simulink model "Powertrain_Comparison"  (R2024b)
settings: Solver=FixedStepDiscrete  StartTime=0.0  StopTime=3600  FixedStep=1  RelTol=1e-3
InitFcn:
  | try; sc=find_system(bdroot,'LookUnderMasks','all','FollowLinks','on','BlockType','Scope'); for k=1:numel(sc); c=get_param(sc{k},'ScopeConfiguration'); try; c.AxesScaling='Auto'; catch; end; try; nd=prod(c.LayoutDimensions); catch; nd=1; end; for d=1:nd; try; c.ActiveDisplay=d; catch; end; try; c.ShowLegend=true; catch; end; end; end; catch; end
(part 1 of 4)
Description:
  | Standalone requested-speed fuel-cell/battery and diesel energy comparison. Repaired with native MATLAB R2024b block ports and connections. Component data remain study assumptions.
settings Model: Creator=Bless Kofi Atisu  LastModifiedBy=Kuami-Neymar
settings ConfigSet: Description=Self-contained HiAce comparison; discrete one-second simulation
settings SolverCC: AlgebraicLoopSolver=TrustRegion
settings DataIOCC: ExternalInput=[]  InitialState=[]  VisualizeSimOutput=off
settings DebuggingCC: SignalInfNanChecking=error  UnconnectedInputMsg=error  UnconnectedOutputMsg=error  UnconnectedLineMsg=error
settings ModelReferenceCC: EnableRefExpFcnMdlSchedulingChecks=on
settings RTWCC: GPUComputeCapability=3.5  DLArmComputeVersion=19.05

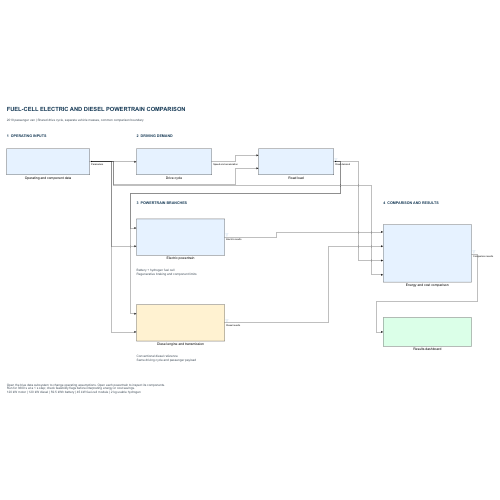
[thumbnail: Simulink's stored preview of the top-level diagram]
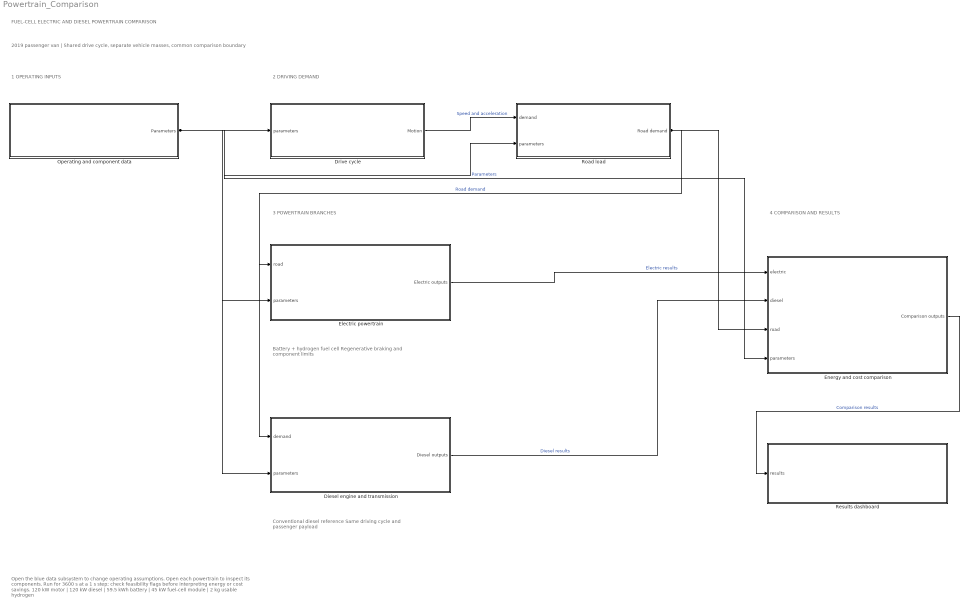
== system Powertrain_Comparison ==
  note: FUEL-CELL ELECTRIC AND DIESEL POWERTRAIN COMPARISON
  note: 2019 passenger van | Shared drive cycle, separate vehicle masses, common comparison boundary
  note: 1 OPERATING INPUTS
  note: 2 DRIVING DEMAND
  note: 3 POWERTRAIN BRANCHES
  note: 4 COMPARISON AND RESULTS
  note: Battery + hydrogen fuel cell
      | Regenerative braking and component limits
  note: Conventional diesel reference
      | Same driving cycle and passenger payload
  note: Open the blue data subsystem to change operating assumptions. Open each powertrain to inspect its components.
      | Run for 3600 s at a 1 s step; check feasibility flags before interpreting energy or cost savings.
      | 120 kW motor | 120 kW diesel | 59.5 kWh battery | 45 kW fuel-cell module | 2 kg usable hydrogen
  Diesel engine and transmission : Subsystem
  Drive cycle : Subsystem
  Electric powertrain : Subsystem
  Energy and cost comparison : Subsystem
  Operating and component data : Subsystem
  Results dashboard : Subsystem
  Road load : Subsystem
  wires:
  Diesel engine and transmission/1(Diesel outputs) -> Energy and cost comparison/2(diesel)  "Diesel results"
  Operating and component data/1(Parameters) -> Road load/2(parameters), Energy and cost comparison/4(parameters), Electric powertrain/2(parameters), Diesel engine and transmission/2(parameters), Drive cycle/1(parameters)  "Parameters"
  Drive cycle/1(Motion) -> Road load/1(demand)  "Speed and acceleration"
  Road load/1(Road demand) -> Energy and cost comparison/3(road), Electric powertrain/1(road), Diesel engine and transmission/1(demand)  "Road demand"
  Energy and cost comparison/1(Comparison outputs) -> Results dashboard/1(results)  "Comparison results"
  Electric powertrain/1(Electric outputs) -> Energy and cost comparison/1(electric)  "Electric results"

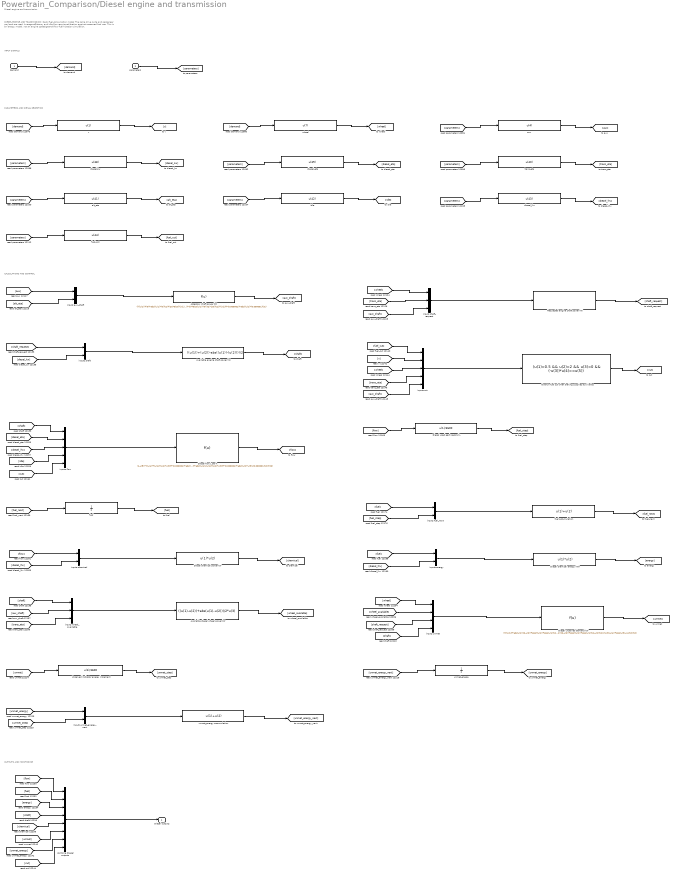
== system Powertrain_Comparison/Diesel engine and transmission ==
  note: Diesel engine and transmission
  note: DIESEL ENGINE AND TRANSMISSION | basic fuel-consumption model
      | The same drive cycle and passenger payload are used. Average efficiency and idle flow require calibration against measured
      | fuel use.
      | This is an energy model, not an engine speed/gear-shift or fuel-injection simulation.
  note: INPUT SIGNALS
  note: PARAMETERS AND SIGNAL SELECTION
  note: CALCULATIONS AND CONTROL
  note: OUTPUTS AND MONITORING
  demand : Inport  PortDimensions=9
  parameters : Inport  Port=2  PortDimensions=52
  Accessory shaft power kW : Fcn  Expr=(((((u(1))+(0)+abs((u(1))-(0)))/2)+(20)-abs((((u(1))+(0)+abs((u(1))-(0)))/2)-(20)))/2)/(((u(2))+(0.000001)+abs((u(2))-(0.000001)))/2)
  Available diesel wheel power kW : Fcn  Expr=((u(1)-u(2))+abs(u(1)-u(2)))/2*u(3)
  Available engine shaft power kW : Fcn  Expr=((u(1))+(u(2))-abs((u(1))-(u(2))))/2
  Diesel chemical energy kWh : Fcn  Expr=u(1)*u(2)
  Diesel chemical power kW : Fcn  Expr=u(1)*u(2)
  Diesel flow L per h : Fcn  Expr=(1-u(5))*(((u(4))+(u(1)/(((u(2)*u(3))+(0.000001)+abs((u(2)*u(3))-(0.000001)))/2))+abs((u(4))-(u(1)/(((u(2)*u(3))+(0.000001)+abs((u(2)*u(3))-(0.000001)))/2))))/2)
  Diesel unserved demand kW : Fcn  Expr=((((((u(1))+abs(u(1)))/2-u(2))+abs(((u(1))+abs(u(1)))/2-u(2)))/2)+(((u(3)-u(4))+abs(u(3)-u(4)))/2)+abs((((((u(1))+abs(u(1)))/2-u(2))+abs(((u(1))+abs(u(1)))/2-u(2)))/2)-(((u(3)-u(4))+abs(u(3)-u(4)))/2)))/2
  Diesel used each second L : Fcn  Expr=u(1)/3600
  Overrun fuel cut when braking supplies auxiliaries : Fcn  Expr=(u(1)>0.5 && u(2)>2 && u(3)<0 && (-u(3))*u(4)>=u(5))
  Requested engine shaft power kW : Fcn  Expr=(((u(1))+abs(u(1)))/2)/(((u(2))+(0.000001)+abs((u(2))-(0.000001)))/2)+u(3)
  Unserved indicator energy increment : Fcn  Expr=u(1)/3600
  alt_eta : Fcn  Expr=u(41)
  aux : Fcn  Expr=u(4)
  combine Diesel outputs : Mux  Inputs=8
  diesel_eta : Fcn  Expr=u(39)
  diesel_kw : Fcn  Expr=u(38)
  diesel_lhv : Fcn  Expr=u(43)
  fuel : UnitDelay
  fuel accumulation : Fcn  Expr=u(1)+u(2)
  fuel_cut : Fcn  Expr=u(44)
  idle : Fcn  Expr=u(42)
  inputs aux_shaft : Mux  Inputs=2
  inputs chemical : Mux  Inputs=2
  inputs cut : Mux  Inputs=5
  inputs energy : Mux  Inputs=2
  inputs flow : Mux  Inputs=5
  inputs fuel_next : Mux  Inputs=2
  inputs shaft : Mux  Inputs=2
  inputs shaft_request : Mux  Inputs=3
  inputs unmet : Mux
  inputs unmet_energy_next : Mux  Inputs=2
  inputs wheel_available : Mux  Inputs=3
  trans_eta : Fcn  Expr=u(40)
  unmet_energy : UnitDelay
  unmet_energy accumulation : Fcn  Expr=u(1)+u(2)
  v : Fcn  Expr=u(1)
  wheel : Fcn  Expr=u(7)
  Diesel outputs : Outport  PortDimensions=8
  wires:
  [parameters] -> trans_eta/1
  Accessory shaft power kW/1 -> [aux_shaft]
  [parameters] -> idle/1
  [shaft] -> inputs wheel_available/1
  [parameters] -> fuel_cut/1
  [diesel_lhv] -> inputs chemical/2
  [flow] -> inputs chemical/1
  [fuel] -> inputs fuel_next/1
  [energy] -> combine Diesel outputs/3
  [diesel_lhv] -> inputs energy/2
  [flow] -> Diesel used each second L/1
  [diesel_lhv] -> inputs flow/3
  [flow] -> combine Diesel outputs/1
  [parameters] -> diesel_kw/1
  [fuel_next] -> fuel/1
  [idle] -> inputs flow/4
  [fuel] -> combine Diesel outputs/2
  [trans_eta] -> inputs cut/4
  [unmet] -> Unserved indicator energy increment/1
  Overrun fuel cut when braking supplies auxiliaries/1 -> [cut]
  [shaft_request] -> inputs unmet/3
  [shaft] -> combine Diesel outputs/4
  [diesel_kw] -> inputs shaft/2
  [demand] -> wheel/1
  [cut] -> combine Diesel outputs/8
  [chemical] -> combine Diesel outputs/5
  [wheel] -> inputs shaft_request/1
  [unmet_step] -> inputs unmet_energy_next/2
  [unmet] -> combine Diesel outputs/6
  [unmet_energy] -> combine Diesel outputs/7
  parameters/1 -> [parameters]
  [parameters] -> diesel_lhv/1
  [parameters] -> alt_eta/1
  [parameters] -> diesel_eta/1
  [shaft] -> inputs flow/1
  demand/1 -> [demand]
  [demand] -> v/1
  [aux_shaft] -> inputs wheel_available/2
  [cut] -> inputs flow/5
  [diesel_eta] -> inputs flow/2
  [trans_eta] -> inputs shaft_request/2
  [shaft_request] -> inputs shaft/1
  [shaft] -> inputs unmet/4
  [trans_eta] -> inputs wheel_available/3
  Diesel chemical energy kWh/1 -> [energy]
  [fuel] -> inputs energy/1
  [fuel_cut] -> inputs cut/1
  [parameters] -> aux/1
  [fuel_step] -> inputs fuel_next/2
  inputs unmet/1 -> Diesel unserved demand kW/1
  [wheel] -> inputs unmet/1
  inputs fuel_next/1 -> fuel accumulation/1
  inputs shaft_request/1 -> Requested engine shaft power kW/1
  [wheel_available] -> inputs unmet/2
  [wheel] -> inputs cut/3
  [v] -> inputs cut/2
  Diesel unserved demand kW/1 -> [unmet]
  [unmet_energy] -> inputs unmet_energy_next/1
  [unmet_energy_next] -> unmet_energy/1
  [aux_shaft] -> inputs cut/5
  unmet_energy/1 -> [unmet_energy]
  [aux] -> inputs aux_shaft/1
  [aux_shaft] -> inputs shaft_request/3
  [alt_eta] -> inputs aux_shaft/2
  fuel_cut/1 -> [fuel_cut]
  combine Diesel outputs/1 -> Diesel outputs/1
  inputs flow/1 -> Diesel flow L per h/1
  diesel_eta/1 -> [diesel_eta]
  inputs wheel_available/1 -> Available diesel wheel power kW/1
  fuel/1 -> [fuel]
  wheel/1 -> [wheel]
  diesel_kw/1 -> [diesel_kw]
  Unserved indicator energy increment/1 -> [unmet_step]
  inputs unmet_energy_next/1 -> unmet_energy accumulation/1
  aux/1 -> [aux]
  Diesel used each second L/1 -> [fuel_step]
  inputs shaft/1 -> Available engine shaft power kW/1
  v/1 -> [v]
  inputs aux_shaft/1 -> Accessory shaft power kW/1
  idle/1 -> [idle]
  alt_eta/1 -> [alt_eta]
  inputs cut/1 -> Overrun fuel cut when braking supplies auxiliaries/1
  inputs energy/1 -> Diesel chemical energy kWh/1
  inputs chemical/1 -> Diesel chemical power kW/1
  diesel_lhv/1 -> [diesel_lhv]
  trans_eta/1 -> [trans_eta]
  Diesel flow L per h/1 -> [flow]
  Available diesel wheel power kW/1 -> [wheel_available]
  fuel accumulation/1 -> [fuel_next]
  unmet_energy accumulation/1 -> [unmet_energy_next]
  Available engine shaft power kW/1 -> [shaft]
  Diesel chemical power kW/1 -> [chemical]
  Requested engine shaft power kW/1 -> [shaft_request]

== system Powertrain_Comparison/Drive cycle ==
  note: Drive cycle
  note: DRIVE CYCLE | same speed and road inputs for both powertrains
      | Cycle mode: 600 s repeated demonstration, ramp 0-80 s, cruise 80-500 s, brake 500-580 s, stop 580-600 s.
  note: INPUT SIGNALS
  note: PARAMETERS AND SIGNAL SELECTION
  note: CALCULATIONS AND CONTROL
  note: OUTPUTS AND MONITORING
  parameters : Inport  PortDimensions=52
  Acceleration cruise braking stop fraction : Fcn  Expr=(u(1)<80)*u(1)/80+(u(1)>=80 && u(1)<500)+(u(1)>=500 && u(1)<580)*(580-u(1))/80
  Commanded acceleration m per s2 : Fcn  Expr=u(1)-u(2)
  Commanded distance increment km : Fcn  Expr=u(1)/1000
  Cycle time s : Fcn  Expr=rem(u(1),600)
  Interval mean speed m per s : Fcn  Expr=(u(1)+u(2))/2
  Limited commanded speed m per s : Fcn  Expr=u(1)+((((u(2)-u(1))+(-u(4))+abs((u(2)-u(1))-(-u(4))))/2)+(u(3))-abs((((u(2)-u(1))+(-u(4))+abs((u(2)-u(1))-(-u(4))))/2)-(u(3))))/2
  Simulation time : DigitalClock
  Target speed m per s : Fcn  Expr=(((((u(1))+(0)+abs((u(1))-(0)))/2)+(100)-abs((((u(1))+(0)+abs((u(1))-(0)))/2)-(100)))/2)*((u(2)>=0.5)*u(3)+(u(2)<0.5))/3.6
  accel : Fcn  Expr=u(50)
  combine Motion : Mux  Inputs=3
  decel : Fcn  Expr=u(51)
  distance : UnitDelay
  distance accumulation : Fcn  Expr=u(1)+u(2)
  inputs a : Mux  Inputs=2
  inputs distance_next : Mux  Inputs=2
  inputs next_speed : Mux
  inputs target : Mux  Inputs=3
  inputs v : Mux  Inputs=2
  old_speed : UnitDelay
  profile : Fcn  Expr=u(2)
  speed : Fcn  Expr=u(1)
  Motion : Outport  PortDimensions=3
  wires:
  [speed] -> inputs target/1
  [old_speed] -> inputs a/2
  [next_speed] -> inputs v/2
  [parameters] -> decel/1
  [shape] -> inputs target/3
  [parameters] -> accel/1
  [old_speed] -> inputs v/1
  [next_speed] -> old_speed/1
  Simulation time/1 -> [time]
  inputs v/1 -> Interval mean speed m per s/1
  [accel] -> inputs next_speed/3
  [distance_next] -> distance/1
  [v] -> Commanded distance increment km/1
  parameters/1 -> [parameters]
  [distance_step] -> inputs distance_next/2
  [profile] -> inputs target/2
  [old_speed] -> inputs next_speed/1
  [parameters] -> profile/1
  [phase] -> Acceleration cruise braking stop fraction/1
  [target] -> inputs next_speed/2
  [parameters] -> speed/1
  [next_speed] -> inputs a/1
  [decel] -> inputs next_speed/4
  [time] -> Cycle time s/1
  [v] -> combine Motion/1
  [distance] -> combine Motion/3
  [a] -> combine Motion/2
  profile/1 -> [profile]
  [distance] -> inputs distance_next/1
  inputs distance_next/1 -> distance accumulation/1
  decel/1 -> [decel]
  accel/1 -> [accel]
  distance/1 -> [distance]
  old_speed/1 -> [old_speed]
  Commanded distance increment km/1 -> [distance_step]
  inputs a/1 -> Commanded acceleration m per s2/1
  speed/1 -> [speed]
  inputs next_speed/1 -> Limited commanded speed m per s/1
  Cycle time s/1 -> [phase]
  inputs target/1 -> Target speed m per s/1
  distance accumulation/1 -> [distance_next]
  combine Motion/1 -> Motion/1
  Acceleration cruise braking stop fraction/1 -> [shape]
  Interval mean speed m per s/1 -> [v]
  Commanded acceleration m per s2/1 -> [a]
  Limited commanded speed m per s/1 -> [next_speed]
  Target speed m per s/1 -> [target]

== system Powertrain_Comparison/Electric powertrain ==
  note: Electric powertrain
  note: ELECTRIC POWERTRAIN | hydrogen and battery feed the electric motor
      | Battery management is reused from the battery project. Motor and converter equations are adapted from the electric-drive
      | project.
  note: INPUT SIGNALS
  note: CALCULATIONS AND CONTROL
  note: OUTPUTS AND MONITORING
  road : Inport  PortDimensions=9
  parameters : Inport  Port=2  PortDimensions=52
  Ambient temperature : Fcn  Expr=u(5)
  Battery DC converter : Subsystem
  Battery power limits : Subsystem
  Battery storage : Subsystem
  DC boost converter : Subsystem
  DC bus and braking : Subsystem
  Energy management : Subsystem
  Fuel cell module : Subsystem
  Hydrogen storage : Subsystem
  Inverter : Subsystem
  Motor : Subsystem
  combine Electric outputs : Mux  Inputs=9
  Electric outputs : Outport  PortDimensions=51
  wires:
  DC bus and braking/1(Bus signals) -> [balance]
  [motor] -> DC bus and braking/4(motor)
  Motor/1(Motor signals) -> [motor], Inverter/1(demand)
  [inverter] -> DC bus and braking/1(inverter)
  [fc_converter] -> DC bus and braking/2(fc_bus)
  [fuelcell] -> Hydrogen storage/1(demand)
  [battery_actual] -> DC bus and braking/3(battery_actual)
  road/1 -> [road]
  [road] -> DC bus and braking/5(road)
  [parameters] -> DC bus and braking/6(parameters)
  DC boost converter/1(Converter signals) -> [fc_converter]
  [parameters] -> Hydrogen storage/2(parameters)
  Battery DC converter/1(Current command) -> [current]
  [ems] -> Battery DC converter/1(dispatch)
  [fc_converter] -> Battery DC converter/2(fuel_cell_bus)
  [battery_state] -> Battery DC converter/3(battery_state)
  [limits] -> Battery DC converter/4(limits)
  [parameters] -> Battery DC converter/5(parameters)
  [road] -> Motor/1(demand)
  [parameters] -> Motor/2(parameters)
  [inverter] -> Energy management/1(inverter)
  [battery_state] -> Energy management/2(battery)
  [limits] -> Energy management/3(limits)
  [hydrogen] -> Energy management/4(hydrogen)
  [parameters] -> Energy management/5(parameters)
  [hydrogen] -> combine Electric outputs/6
  parameters/1 -> [parameters]
  [battery_state] -> Battery power limits/1(demand)
  [parameters] -> Battery power limits/2(parameters)
  Battery storage/1(Battery state) -> [battery_state]
  [parameters] -> Ambient temperature/1
  [battery_state] -> combine Electric outputs/1
  [battery_actual] -> combine Electric outputs/2
  [motor] -> combine Electric outputs/3
  [inverter] -> combine Electric outputs/4
  [fuelcell] -> combine Electric outputs/5
  [fc_converter] -> combine Electric outputs/7
  [balance] -> combine Electric outputs/8
  [battery_request] -> combine Electric outputs/9
  [current] -> Battery storage/1(current_request)
  Hydrogen storage/1(Inventory) -> [hydrogen]
  Ambient temperature/1 -> Battery storage/2(ambient)
  Battery DC converter/2(Converter request) -> [battery_request]
  Energy management/1(Dispatch) -> [ems], Fuel cell module/1(dispatch)
  [parameters] -> Inverter/2(parameters)
  [hydrogen] -> Fuel cell module/2(hydrogen)
  [parameters] -> Fuel cell module/3(parameters)
  Battery power limits/1(Power limits) -> [limits]
  combine Electric outputs/1 -> Electric outputs/1
  Inverter/1(Inverter signals) -> [inverter]
  Battery storage/2(Battery actual) -> [battery_actual]
  Fuel cell module/1(Fuel cell signals) -> DC boost converter/1(demand), [fuelcell]
  [parameters] -> DC boost converter/2(parameters)

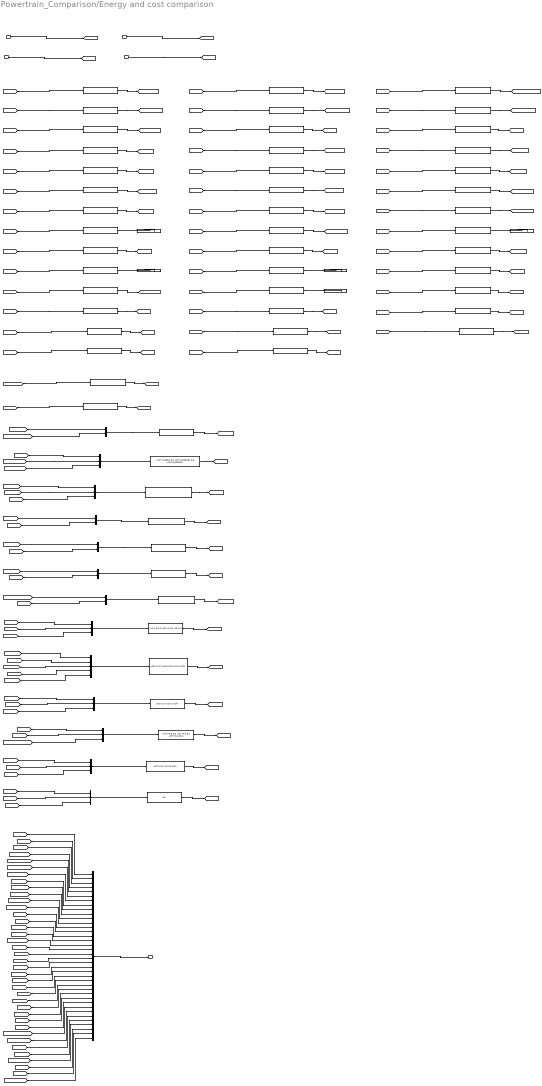
== system Powertrain_Comparison/Energy and cost comparison ==
  note: Energy and cost comparison
  note: ENERGY AND COST COMPARISON | common requested route and payload
      | Net source energy = hydrogen LHV energy + signed battery inventory depletion. Fuel-cell electricity is not counted again.
      | Saving outputs are valid only if both powertrains meet demand. Cost savings also require prices and no battery-energy
      | surplus.
  note: INPUT SIGNALS
  note: PARAMETERS AND SIGNAL SELECTION
  note: CALCULATIONS AND CONTROL
  note: OUTPUTS AND MONITORING
  electric : Inport  PortDimensions=51
  diesel : Inport  Port=2  PortDimensions=8
  road : Inport  Port=3  PortDimensions=9
  parameters : Inport  Port=4  PortDimensions=52
  All energy prices entered 1 yes : Fcn  Expr=(u(1)>0 && u(2)>0 && u(3)>0)
  Battery SOC percent : Fcn  Expr=100*u(1)
  Both powertrains support requested operation 1 yes : Fcn  Expr=(u(1)>0.0001 && u(2)<0.000001 && u(3)<0.000001)
  Calculated diesel litres per 100 km : Fcn  Expr=100*u(1)/(((u(2))+(0.000001)+abs((u(2))-(0.000001)))/2)
  Commanded speed km per h : Fcn  Expr=3.6*u(1)
  Cost saving comparison valid 1 yes : Fcn  Expr=(u(1)>0.5 && u(2)>0.5 && u(3)>=-0.001)
  Diesel refill cost GHS : Fcn  Expr=u(3)*u(1)*u(2)-(1-u(3))
  Energy cost saving GHS -1 unavailable : Fcn  Expr=u(3)*(u(1)-u(2))-(1-u(3))
  Grid recharge energy equivalent kWh : Fcn  Expr=((u(1))+abs(u(1)))/2/(((u(2))+(0.000001)+abs((u(2))-(0.000001)))/2)
  Hydrogen kg per 100 km : Fcn  Expr=100*u(1)/(((u(2))+(0.000001)+abs((u(2))-(0.000001)))/2)
  Hydrogen refill plus recharge cost GHS : Fcn  Expr=u(5)*(u(1)*u(2)+u(3)*u(4))-(1-u(5))
  Mass above study screen kg : Fcn  Expr=((((u(1))+(u(2))+abs((u(1))-(u(2))))/2-u(3))+abs(((u(1))+(u(2))+abs((u(1))-(u(2))))/2-u(3)))/2
  Net onboard source energy kWh : Fcn  Expr=u(1)+u(2)
  Net source energy kWh per 100 km : Fcn  Expr=100*u(1)/(((u(2))+(0.000001)+abs((u(2))-(0.000001)))/2)
  Net source energy saving percent -1 unavailable : Fcn  Expr=u(3)*100*(1-u(1)/(((u(2))+(0.000001)+abs((u(2))-(0.000001)))/2))-(1-u(3))
  Unused diagnostic balance_friction : Terminator
  Unused diagnostic balance_load_energy : Terminator
  Unused diagnostic diesel_chemical : Terminator
  Unused diagnostic diesel_cut : Terminator
  Unused diagnostic diesel_shaft : Terminator
  balance_battery_bus : Fcn  Expr=u(40)
  balance_friction : Fcn  Expr=u(45)
  balance_load_energy : Fcn  Expr=u(47)
  balance_regen_energy : Fcn  Expr=u(48)
  balance_regen_used : Fcn  Expr=u(42)
  balance_unmet : Fcn  Expr=u(41)
  balance_unmet_energy : Fcn  Expr=u(46)
  battery_actual_current : Fcn  Expr=u(14)
  battery_actual_heat : Fcn  Expr=u(18)
  battery_actual_voltage : Fcn  Expr=u(13)
  battery_state_delta_energy : Fcn  Expr=u(10)
  battery_state_nominal : Fcn  Expr=u(8)
  battery_state_soc : Fcn  Expr=u(1)
  battery_state_temp : Fcn  Expr=u(2)
  combine Comparison outputs : Mux  Inputs=38
  diesel_chemical : Fcn  Expr=u(5)
  diesel_cut : Fcn  Expr=u(8)
  diesel_energy : Fcn  Expr=u(3)
  diesel_flow : Fcn  Expr=u(1)
  diesel_fuel : Fcn  Expr=u(2)
  diesel_price : Fcn  Expr=u(47)
  diesel_shaft : Fcn  Expr=u(4)
  diesel_unmet : Fcn  Expr=u(6)
  diesel_unmet_energy : Fcn  Expr=u(7)
  distance : Fcn  Expr=u(3)
  eta_grid : Fcn  Expr=u(48)
  fc_converter_bus : Fcn  Expr=u(37)
  fuelcell_heat : Fcn  Expr=u(33)
  fuelcell_module : Fcn  Expr=u(31)
  grid_price : Fcn  Expr=u(45)
  gross : Fcn  Expr=u(49)
  h2_price : Fcn  Expr=u(46)
  hydrogen_energy : Fcn  Expr=u(36)
  hydrogen_remaining : Fcn  Expr=u(34)
  hydrogen_used : Fcn  Expr=u(35)
  inputs cost_save : Mux  Inputs=3
  inputs cost_valid : Mux  Inputs=3
  inputs diesel_cost : Mux  Inputs=3
  inputs diesel_l100 : Mux  Inputs=2
  inputs energy_save : Mux  Inputs=3
  inputs ev_cost : Mux  Inputs=5
  inputs ev_kwh100 : Mux  Inputs=2
  inputs feasible : Mux  Inputs=3
  inputs grid_recharge : Mux  Inputs=2
  inputs h2_kg100 : Mux  Inputs=2
  inputs mass_excess : Mux  Inputs=3
  inputs net_ev_energy : Mux  Inputs=2
  inputs prices_ready : Mux  Inputs=3
  mass_ev : Fcn  Expr=u(8)
  mass_ice : Fcn  Expr=u(9)
  motor_iq : Fcn  Expr=u(25)
  motor_phase_v : Fcn  Expr=u(26)
  motor_rpm : Fcn  Expr=u(24)
  motor_unmet_motor : Fcn  Expr=u(27)
  v : Fcn  Expr=u(1)
  Comparison outputs : Outport  PortDimensions=38
  wires:
  [ev_cost] -> combine Comparison outputs/27
  [parameters] -> h2_price/1
  motor_rpm/1 -> [motor_rpm]
  [gross] -> inputs mass_excess/3
  [speed_kmh] -> combine Comparison outputs/1
  combine Comparison outputs/1 -> Comparison outputs/1
  balance_battery_bus/1 -> [balance_battery_bus]
  [battery_state_nominal] -> combine Comparison outputs/32
  [balance_regen_energy] -> combine Comparison outputs/38
  Energy cost saving GHS -1 unavailable/1 -> [cost_save]
  battery_state_delta_energy/1 -> [battery_state_delta_energy]
  [diesel_fuel] -> combine Comparison outputs/20
  [fc_converter_bus] -> combine Comparison outputs/10
  [parameters] -> eta_grid/1
  [fuelcell_heat] -> combine Comparison outputs/34
  [h2_kg100] -> combine Comparison outputs/36
  [ev_kwh100] -> combine Comparison outputs/37
  [diesel] -> diesel_fuel/1
  [ev_cost] -> inputs cost_save/2
  [grid_recharge] -> combine Comparison outputs/26
  [soc_percent] -> combine Comparison outputs/3
  inputs ev_cost/1 -> Hydrogen refill plus recharge cost GHS/1
  Hydrogen kg per 100 km/1 -> [h2_kg100]
  [battery_actual_heat] -> combine Comparison outputs/35
  [net_ev_energy] -> combine Comparison outputs/22
  [mass_excess] -> combine Comparison outputs/33
  [hydrogen_remaining] -> combine Comparison outputs/7
  h2_price/1 -> [h2_price]
  [distance] -> combine Comparison outputs/2
  [battery_state_delta_energy] -> combine Comparison outputs/31
  diesel_flow/1 -> [diesel_flow]
  [mass_ev] -> inputs mass_excess/1
  gross/1 -> [gross]
  [cost_valid] -> combine Comparison outputs/30
  [fuelcell_module] -> combine Comparison outputs/9
  [cost_save] -> combine Comparison outputs/29
  balance_unmet_energy/1 -> [balance_unmet_energy]
  [diesel_cost] -> combine Comparison outputs/28
  [diesel_price] -> inputs diesel_cost/2
  [energy_save] -> combine Comparison outputs/24
  [net_ev_energy] -> inputs ev_kwh100/1
  Diesel refill cost GHS/1 -> [diesel_cost]
  mass_ice/1 -> [mass_ice]
  [diesel] -> diesel_cut/1
  [diesel_l100] -> combine Comparison outputs/21
  [balance_regen_used] -> combine Comparison outputs/12
  [electric] -> motor_iq/1
  [battery_actual_voltage] -> combine Comparison outputs/5
  [motor_unmet_motor] -> combine Comparison outputs/17
  [prices_ready] -> inputs diesel_cost/3
  [feasible] -> combine Comparison outputs/25
  balance_load_energy/1 -> Unused diagnostic balance_load_energy/1
  [diesel_unmet] -> combine Comparison outputs/18
  parameters/1 -> [parameters]
  [battery_actual_current] -> combine Comparison outputs/6
  [distance] -> inputs h2_kg100/2
  [battery_state_delta_energy] -> inputs grid_recharge/1
  [diesel_energy] -> combine Comparison outputs/23
  [diesel_flow] -> combine Comparison outputs/19
  diesel/1 -> [diesel]
  [balance_unmet] -> combine Comparison outputs/16
  [motor_phase_v] -> combine Comparison outputs/15
  [motor_iq] -> combine Comparison outputs/14
  balance_regen_used/1 -> [balance_regen_used]
  [battery_state_delta_energy] -> inputs cost_valid/3
  [motor_rpm] -> combine Comparison outputs/13
  [balance_battery_bus] -> combine Comparison outputs/11
  inputs cost_save/1 -> Energy cost saving GHS -1 unavailable/1
  [hydrogen_used] -> combine Comparison outputs/8
  [battery_state_temp] -> combine Comparison outputs/4
  [grid_recharge] -> inputs ev_cost/1
  [diesel] -> diesel_unmet/1
  Mass above study screen kg/1 -> [mass_excess]
  inputs mass_excess/1 -> Mass above study screen kg/1
  [mass_ice] -> inputs mass_excess/2
  [cost_valid] -> inputs cost_save/3
  [diesel_cost] -> inputs cost_save/1
  [battery_state_delta_energy] -> inputs net_ev_energy/2
  Cost saving comparison valid 1 yes/1 -> [cost_valid]
  [diesel_fuel] -> inputs diesel_cost/1
  inputs cost_valid/1 -> Cost saving comparison valid 1 yes/1
  [prices_ready] -> inputs cost_valid/2
  [road] -> mass_ice/1
  [feasible] -> inputs cost_valid/1
  inputs diesel_cost/1 -> Diesel refill cost GHS/1
  [prices_ready] -> inputs ev_cost/5
  Hydrogen refill plus recharge cost GHS/1 -> [ev_cost]
  [h2_price] -> inputs ev_cost/4
  motor_unmet_motor/1 -> [motor_unmet_motor]
  [hydrogen_used] -> inputs ev_cost/3
  [grid_price] -> inputs ev_cost/2
  All energy prices entered 1 yes/1 -> [prices_ready]
  inputs prices_ready/1 -> All energy prices entered 1 yes/1
  [diesel_price] -> inputs prices_ready/3
  [h2_price] -> inputs prices_ready/2
  fuelcell_heat/1 -> [fuelcell_heat]
  [grid_price] -> inputs prices_ready/1
  Grid recharge energy equivalent kWh/1 -> [grid_recharge]
  inputs grid_recharge/1 -> Grid recharge energy equivalent kWh/1
  [eta_grid] -> inputs grid_recharge/2
  [diesel] -> diesel_energy/1
  Net source energy kWh per 100 km/1 -> [ev_kwh100]
  inputs ev_kwh100/1 -> Net source energy kWh per 100 km/1
  [distance] -> inputs ev_kwh100/2
  fc_converter_bus/1 -> [fc_converter_bus]
  inputs h2_kg100/1 -> Hydrogen kg per 100 km/1
  [hydrogen_used] -> inputs h2_kg100/1
  Calculated diesel litres per 100 km/1 -> [diesel_l100]
  inputs diesel_l100/1 -> Calculated diesel litres per 100 km/1
  battery_actual_heat/1 -> [battery_actual_heat]
  [distance] -> inputs diesel_l100/2
  [diesel_fuel] -> inputs diesel_l100/1
  Net source energy saving percent -1 unavailable/1 -> [energy_save]
  inputs energy_save/1 -> Net source energy saving percent -1 unavailable/1
  [feasible] -> inputs energy_save/3
  [diesel_energy] -> inputs energy_save/2
  [net_ev_energy] -> inputs energy_save/1
  Both powertrains support requested operation 1 yes/1 -> [feasible]
  inputs feasible/1 -> Both powertrains support requested operation 1 yes/1
  battery_state_soc/1 -> [battery_state_soc]
  [diesel_unmet_energy] -> inputs feasible/3
  [balance_unmet_energy] -> inputs feasible/2
  [distance] -> inputs feasible/1
  Net onboard source energy kWh/1 -> [net_ev_energy]
  [parameters] -> gross/1
  inputs net_ev_energy/1 -> Net onboard source energy kWh/1
  [hydrogen_energy] -> inputs net_ev_energy/1
  Commanded speed km per h/1 -> [speed_kmh]
  [v] -> Commanded speed km per h/1
  Battery SOC percent/1 -> [soc_percent]
  [battery_state_soc] -> Battery SOC percent/1
  eta_grid/1 -> [eta_grid]
  diesel_price/1 -> [diesel_price]
  [parameters] -> diesel_price/1
  grid_price/1 -> [grid_price]
  [parameters] -> grid_price/1
  mass_ev/1 -> [mass_ev]
  motor_phase_v/1 -> [motor_phase_v]
  [road] -> mass_ev/1
  distance/1 -> [distance]
  [road] -> distance/1
  v/1 -> [v]
  [road] -> v/1
  diesel_cut/1 -> Unused diagnostic diesel_cut/1
  diesel_unmet_energy/1 -> [diesel_unmet_energy]
  [diesel] -> diesel_chemical/1
  [diesel] -> diesel_unmet_energy/1
  diesel_unmet/1 -> [diesel_unmet]
  diesel_chemical/1 -> Unused diagnostic diesel_chemical/1
  electric/1 -> [electric]
  diesel_shaft/1 -> Unused diagnostic diesel_shaft/1
  [diesel] -> diesel_flow/1
  [diesel] -> diesel_shaft/1
  diesel_energy/1 -> [diesel_energy]
  diesel_fuel/1 -> [diesel_fuel]
  balance_friction/1 -> Unused diagnostic balance_friction/1
  [electric] -> balance_friction/1
  balance_regen_energy/1 -> [balance_regen_energy]
  [electric] -> balance_regen_energy/1
  battery_actual_voltage/1 -> [battery_actual_voltage]
  [electric] -> balance_load_energy/1
  motor_iq/1 -> [motor_iq]
  [electric] -> balance_unmet_energy/1
  [electric] -> balance_regen_used/1
  balance_unmet/1 -> [balance_unmet]
  [electric] -> balance_unmet/1
  [electric] -> balance_battery_bus/1
  [electric] -> battery_actual_current/1
  [electric] -> fc_converter_bus/1
  hydrogen_energy/1 -> [hydrogen_energy]
  [electric] -> hydrogen_energy/1
  hydrogen_used/1 -> [hydrogen_used]
  [electric] -> hydrogen_used/1
  hydrogen_remaining/1 -> [hydrogen_remaining]
  [electric] -> hydrogen_remaining/1
  [electric] -> fuelcell_heat/1
  fuelcell_module/1 -> [fuelcell_module]
  [electric] -> fuelcell_module/1
  [electric] -> motor_unmet_motor/1
  [electric] -> motor_phase_v/1
  [electric] -> motor_rpm/1
  [electric] -> battery_actual_heat/1
  battery_actual_current/1 -> [battery_actual_current]
  [electric] -> battery_actual_voltage/1
  battery_state_nominal/1 -> [battery_state_nominal]
  [electric] -> battery_state_nominal/1
  [electric] -> battery_state_delta_energy/1
  battery_state_temp/1 -> [battery_state_temp]
  [electric] -> battery_state_temp/1
  [electric] -> battery_state_soc/1
  road/1 -> [road]

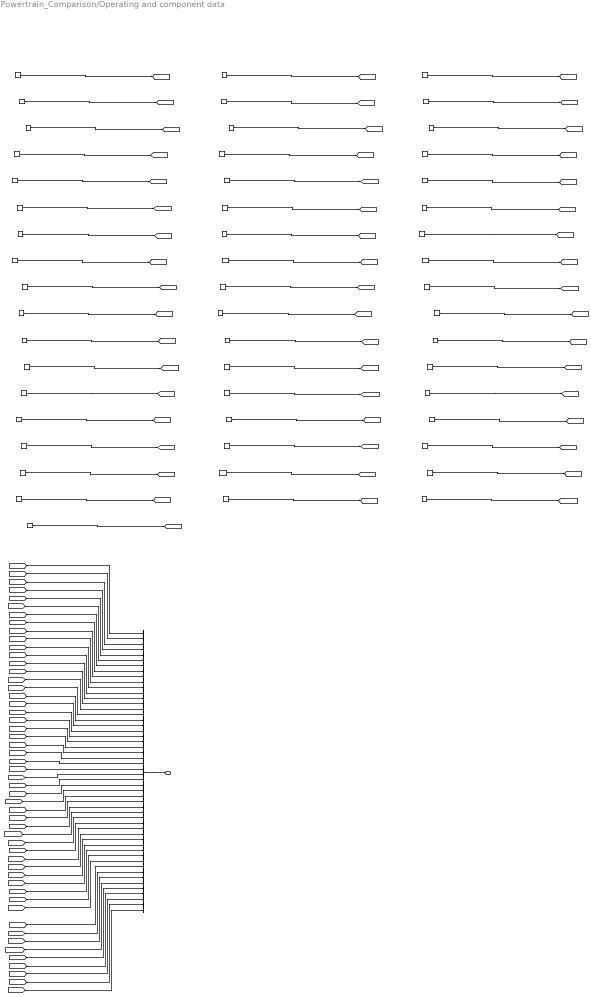
== system Powertrain_Comparison/Operating and component data ==
  note: Operating and component data
  note: ENERGY PRICES
  note: DIESEL ENGINE
  note: FUEL CELL
  note: ELECTRIC DRIVE
  note: VEHICLE DATA
  note: OPERATING CONDITIONS
  note: EDIT PARAMETERS | blue blocks hold numeric values inside this file
      | Battery cell configuration, initial SOC and thermal values are in Battery storage > Battery management. Stop before editing
      | ratings.
  note: EDITABLE OPERATING AND COMPONENT DATA
  note: OUTPUTS AND MONITORING
  Air density kg per m3 : Constant  Value=1.18
  Alternator efficiency : Constant  Value=0.65
  Ambient temperature deg C : Constant  Value=30
  Auxiliary electrical load kW : Constant  Value=3
  Bidirectional battery converter efficiency : Constant  Value=0.97
  Common passengers and luggage kg : Constant  Value=540
  Converted kerb mass kg : Constant  Value=3004
  Delivered hydrogen GHS per kg : Constant  Value=0
  Diesel GHS per litre : Constant  Value=0
  Diesel LHV kWh per litre : Constant  Value=9.947693
  Diesel average brake efficiency : Constant  Value=0.33
  Diesel engine rated shaft power kW : Constant  Value=120
  Diesel idle fuel rate L per h : Constant  Value=0.8
  Diesel kerb mass kg : Constant  Value=2650
  Diesel transmission efficiency : Constant  Value=0.9
  Drag area CdA m2 : Constant  Value=1.8
  Electric gearbox efficiency : Constant  Value=0.97
  Electric reduction ratio : Constant  Value=10
  Electricity GHS per kWh : Constant  Value=0
  Fuel cell OFF threshold percent : Constant  Value=80
  Fuel cell ON threshold percent : Constant  Value=60
  Fuel cell boost converter efficiency : Constant  Value=0.95
  Fuel cell charging allowance kW : Constant  Value=10
  Fuel cell enable 1 or 0 : Constant
  Fuel cell module ramp kW per s : Constant  Value=2
  Fuel cell module rated output kW : Constant  Value=45
  Fuel cell net electrical efficiency LHV : Constant  Value=0.5
  Fuel cell nominal output voltage V : Constant  Value=300
  Grid to stored battery charging efficiency : Constant  Value=0.92
  Gross mass screen kg : Constant  Value=3710
  Hydrogen LHV kWh per kg : Constant  Value=33.3
  Initial usable hydrogen kg : Constant  Value=2
  Inverter efficiency : Constant  Value=0.97
  Loaded wheel radius m : Constant  Value=0.35
  Maximum modulation index : Constant  Value=0.95
  Maximum requested acceleration m per s2 : Constant
  Maximum requested deceleration m per s2 : Constant
  Motor PM flux Wb : Constant  Value=0.08
  Motor dq peak current A : Constant  Value=625
  Motor peak shaft power kW : Constant  Value=120
  Motor peak shaft torque Nm : Constant  Value=300
  Motor pole pairs : Constant  Value=4
  Motor viscous damping Nm s per rad : Constant  Value=0.001
  Overrun fuel cut enable 1 or 0 : Constant
  Profile 1 cycle 0 constant : Constant
  Regenerative wheel power limit kW : Constant  Value=60
  Regulated DC link voltage V : Constant  Value=600
  Road gradient percent : Constant  Value=0
  Rolling resistance coefficient : Constant  Value=0.012
  Scaled dq inductance H : Constant  Value=6.4e-05
  Scaled phase resistance ohm : Constant  Value=0.0064
  Target speed km per h : Constant  Value=80
  combine Parameters : Mux  Inputs=52
  Parameters : Outport  PortDimensions=52
  wires:
  Fuel cell charging allowance kW/1 -> [charge_boost]
  Diesel transmission efficiency/1 -> [trans_eta]
  Ambient temperature deg C/1 -> [ambient]
  Electric reduction ratio/1 -> [gear]
  Diesel idle fuel rate L per h/1 -> [idle]
  Bidirectional battery converter efficiency/1 -> [eta_bconv]
  Maximum requested deceleration m per s2/1 -> [decel]
  Regenerative wheel power limit kW/1 -> [regen_kw]
  Auxiliary electrical load kW/1 -> [aux]
  Diesel engine rated shaft power kW/1 -> [diesel_kw]
  [ambient] -> combine Parameters/5
  Scaled dq inductance H/1 -> [lq]
  Fuel cell module ramp kW per s/1 -> [fc_ramp]
  Overrun fuel cut enable 1 or 0/1 -> [fuel_cut]
  [ice_kerb] -> combine Parameters/8
  Rolling resistance coefficient/1 -> [crr]
  [grade] -> combine Parameters/3
  Motor viscous damping Nm s per rad/1 -> [b]
  Converted kerb mass kg/1 -> [ev_kerb]
  Loaded wheel radius m/1 -> [radius]
  Diesel GHS per litre/1 -> [diesel_price]
  Diesel LHV kWh per litre/1 -> [diesel_lhv]
  Diesel average brake efficiency/1 -> [diesel_eta]
  Fuel cell net electrical efficiency LHV/1 -> [eta_fc]
  Initial usable hydrogen kg/1 -> [h2_initial]
  Inverter efficiency/1 -> [eta_inv]
  Diesel kerb mass kg/1 -> [ice_kerb]
  Fuel cell nominal output voltage V/1 -> [fc_voltage]
  Hydrogen LHV kWh per kg/1 -> [h2_lhv]
  [imax] -> combine Parameters/23
  [aux] -> combine Parameters/4
  Scaled phase resistance ohm/1 -> [rs]
  Fuel cell module rated output kW/1 -> [fc_kw]
  Road gradient percent/1 -> [grade]
  Electric gearbox efficiency/1 -> [eta_gear]
  Delivered hydrogen GHS per kg/1 -> [h2_price]
  Electricity GHS per kWh/1 -> [grid_price]
  [eta_gear] -> combine Parameters/15
  [speed] -> combine Parameters/1
  [profile] -> combine Parameters/2
  [fc_enable] -> combine Parameters/6
  [crr] -> combine Parameters/12
  [payload] -> combine Parameters/7
  [vbus] -> combine Parameters/25
  [ev_kerb] -> combine Parameters/9
  [rho] -> combine Parameters/10
  [mod] -> combine Parameters/24
  [cda] -> combine Parameters/11
  [radius] -> combine Parameters/13
  [gear] -> combine Parameters/14
  [motor_kw] -> combine Parameters/16
  [torque] -> combine Parameters/17
  [pole] -> combine Parameters/18
  [flux] -> combine Parameters/19
  [eta_bconv] -> combine Parameters/27
  [rs] -> combine Parameters/20
  [b] -> combine Parameters/22
  [lq] -> combine Parameters/21
  [eta_inv] -> combine Parameters/26
  [fc_kw] -> combine Parameters/28
  [eta_fc] -> combine Parameters/29
  [soc_on] -> combine Parameters/32
  [eta_fcconv] -> combine Parameters/30
  [fc_ramp] -> combine Parameters/31
  [soc_off] -> combine Parameters/33
  [charge_boost] -> combine Parameters/34
  [h2_initial] -> combine Parameters/35
  [h2_lhv] -> combine Parameters/36
  [regen_kw] -> combine Parameters/37
  [diesel_kw] -> combine Parameters/38
  [diesel_eta] -> combine Parameters/39
  [trans_eta] -> combine Parameters/40
  [alt_eta] -> combine Parameters/41
  [idle] -> combine Parameters/42
  [diesel_lhv] -> combine Parameters/43
  [fuel_cut] -> combine Parameters/44
  [grid_price] -> combine Parameters/45
  [h2_price] -> combine Parameters/46
  [diesel_price] -> combine Parameters/47
  [eta_grid] -> combine Parameters/48
  [gross] -> combine Parameters/49
  [accel] -> combine Parameters/50
  [decel] -> combine Parameters/51
  [fc_voltage] -> combine Parameters/52
  Fuel cell enable 1 or 0/1 -> [fc_enable]
  Air density kg per m3/1 -> [rho]
  Common passengers and luggage kg/1 -> [payload]
  Maximum requested acceleration m per s2/1 -> [accel]
  Maximum modulation index/1 -> [mod]
  Motor peak shaft power kW/1 -> [motor_kw]
  Profile 1 cycle 0 constant/1 -> [profile]
  Motor peak shaft torque Nm/1 -> [torque]
  Regulated DC link voltage V/1 -> [vbus]
  Grid to stored battery charging efficiency/1 -> [eta_grid]
  Fuel cell ON threshold percent/1 -> [soc_on]
  Fuel cell OFF threshold percent/1 -> [soc_off]
  Motor PM flux Wb/1 -> [flux]
  Target speed km per h/1 -> [speed]
  Gross mass screen kg/1 -> [gross]
  Alternator efficiency/1 -> [alt_eta]
  Fuel cell boost converter efficiency/1 -> [eta_fcconv]
  Motor dq peak current A/1 -> [imax]
  Motor pole pairs/1 -> [pole]
  Drag area CdA m2/1 -> [cda]
  combine Parameters/1 -> Parameters/1

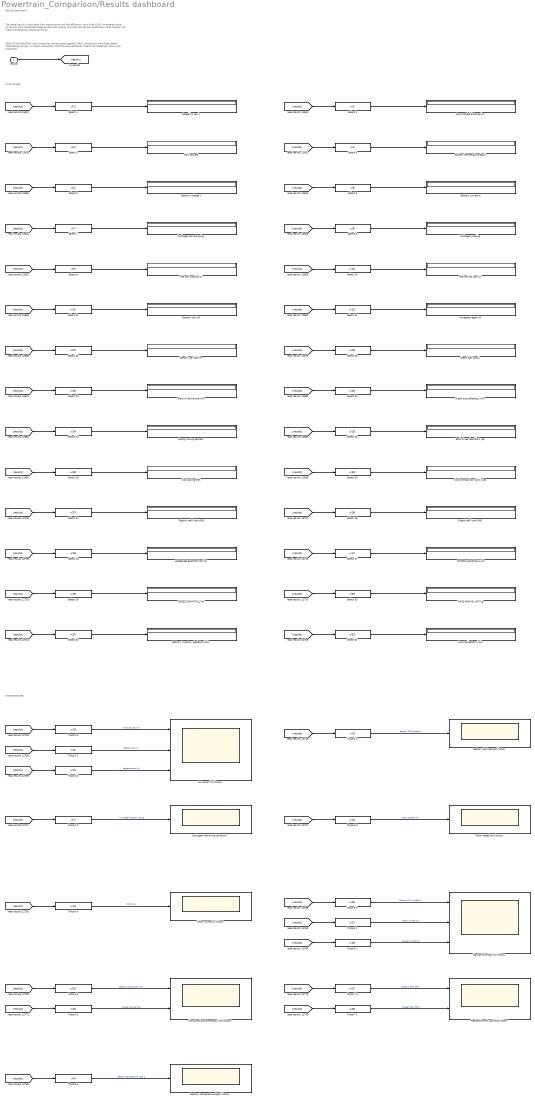
== system Powertrain_Comparison/Results dashboard ==
  note: Results dashboard
  note: The diesel result is calculated from engine power and fuel efficiency, not a fixed L/100 km entered value.
      | All results are a requested-speed assessment. Energy and cost savings are conditional model outputs, not measured Ghanaian
      | operating results.
  note: RESULTS DASHBOARD | each Scope has named signal legends
      | Check comparison-valid flags before interpreting savings. -1 means unavailable. Positive unserved power means the requested
      | route is not supported.
  note: LIVE VALUES
  note: TIME HISTORIES
  results : Inport  PortDimensions=38
  Accepted regen kW : Display
  Battery SOC percent history : Scope
  Battery bus kW : Display
  Battery current A : Display
  Battery inventory depletion kWh : Display
  Battery temperature deg C : Display
  Battery temperature deg C history : Scope
  Battery voltage V : Display
  Both drives feasible 1 yes : Display
  Commanded distance km : Display
  Consumed source energy kWh history : Scope  NumInputPorts=2
  Cost comparison valid 1 yes : Display
  Cost saving GHS : Display
  DC power kW history : Scope  NumInputPorts=3
  DIESEL SHORTFALL kW : Display
  Demand shortfall kW history : Scope  NumInputPorts=3
  Diesel L per 100 km : Display
  Diesel fuel used L : Display
  Diesel refill cost GHS : Display
  Diesel source energy kWh : Display
  Electric net source kWh : Display
  Electric refill cost GHS : Display
  Energy saving percent : Display
  Fuel cell DC bus kW : Display
  Fuel cell module kW : Display
  Hydrogen remaining kg : Display
  Hydrogen remaining kg history : Scope
  Hydrogen used kg : Display
  MASS ABOVE LIMIT kg : Display
  MOTOR SHORTFALL kW : Display
  Motor current A history : Scope
  Motor speed rpm history : Scope
  Nominal battery kWh : Display
  Replenishment cost GHS history : Scope  NumInputPorts=2
  SOC percent : Display
  Select 1 : Fcn  Expr=u(1)
  Select 10 : Fcn  Expr=u(10)
  Select 11 : Fcn  Expr=u(11)
  Select 12 : Fcn  Expr=u(12)
  Select 16 : Fcn  Expr=u(16)
  Select 17 : Fcn  Expr=u(17)
  Select 18 : Fcn  Expr=u(18)
  Select 2 : Fcn  Expr=u(2)
  Select 20 : Fcn  Expr=u(20)
  Select 21 : Fcn  Expr=u(21)
  Select 22 : Fcn  Expr=u(22)
  Select 23 : Fcn  Expr=u(23)
  Select 24 : Fcn  Expr=u(24)
  Select 25 : Fcn  Expr=u(25)
  Select 27 : Fcn  Expr=u(27)
  Select 28 : Fcn  Expr=u(28)
  Select 29 : Fcn  Expr=u(29)
  Select 3 : Fcn  Expr=u(3)
  Select 30 : Fcn  Expr=u(30)
  Select 31 : Fcn  Expr=u(31)
  Select 32 : Fcn  Expr=u(32)
  Select 33 : Fcn  Expr=u(33)
  Select 4 : Fcn  Expr=u(4)
  Select 5 : Fcn  Expr=u(5)
  Select 6 : Fcn  Expr=u(6)
  Select 7 : Fcn  Expr=u(7)
  Select 8 : Fcn  Expr=u(8)
  Select 9 : Fcn  Expr=u(9)
  Speed km per h : Display
  Trace 0 0 : Fcn  Expr=u(10)
  Trace 0 1 : Fcn  Expr=u(11)
  Trace 0 2 : Fcn  Expr=u(12)
  Trace 1 0 : Fcn  Expr=u(3)
  Trace 2 0 : Fcn  Expr=u(7)
  Trace 3 0 : Fcn  Expr=u(13)
  Trace 4 0 : Fcn  Expr=u(14)
  Trace 5 0 : Fcn  Expr=u(16)
  Trace 5 1 : Fcn  Expr=u(17)
  Trace 5 2 : Fcn  Expr=u(18)
  Trace 6 0 : Fcn  Expr=u(22)
  Trace 6 1 : Fcn  Expr=u(23)
  Trace 7 0 : Fcn  Expr=u(27)
  Trace 7 1 : Fcn  Expr=u(28)
  Trace 8 0 : Fcn  Expr=u(4)
  UNSERVED ELECTRIC DC kW : Display
  wires:
  Select 12/1 -> Accepted regen kW/1
  Trace 1 0/1 -> Battery SOC percent history/1  "Battery SOC percent"
  Select 11/1 -> Battery bus kW/1
  Select 6/1 -> Battery current A/1
  Select 31/1 -> Battery inventory depletion kWh/1
  Select 4/1 -> Battery temperature deg C/1
  Trace 8 0/1 -> Battery temperature deg C history/1  "Battery temperature deg C"
  Select 5/1 -> Battery voltage V/1
  Select 25/1 -> Both drives feasible 1 yes/1
  Select 2/1 -> Commanded distance km/1
  Trace 6 0/1 -> Consumed source energy kWh history/1  "Electric net source kWh"
  Trace 6 1/1 -> Consumed source energy kWh history/2  "Diesel source kWh"
  Select 30/1 -> Cost comparison valid 1 yes/1
  Select 29/1 -> Cost saving GHS/1
  Trace 0 0/1 -> DC power kW history/1  "Fuel cell DC kW"
  Trace 0 1/1 -> DC power kW history/2  "Battery DC kW"
  Trace 0 2/1 -> DC power kW history/3  "Regeneration kW"
  Select 18/1 -> DIESEL SHORTFALL kW/1
  Trace 5 0/1 -> Demand shortfall kW history/1  "Electric DC unmet kW"
  Trace 5 1/1 -> Demand shortfall kW history/2  "Motor unmet kW"
  Trace 5 2/1 -> Demand shortfall kW history/3  "Diesel unmet kW"
  Select 21/1 -> Diesel L per 100 km/1
  Select 20/1 -> Diesel fuel used L/1
  Select 28/1 -> Diesel refill cost GHS/1
  Select 23/1 -> Diesel source energy kWh/1
  Select 22/1 -> Electric net source kWh/1
  Select 27/1 -> Electric refill cost GHS/1
  Select 24/1 -> Energy saving percent/1
  Select 10/1 -> Fuel cell DC bus kW/1
  Select 9/1 -> Fuel cell module kW/1
  Select 7/1 -> Hydrogen remaining kg/1
  Trace 2 0/1 -> Hydrogen remaining kg history/1  "Hydrogen remaining kg"
  Select 8/1 -> Hydrogen used kg/1
  Select 33/1 -> MASS ABOVE LIMIT kg/1
  Select 17/1 -> MOTOR SHORTFALL kW/1
  Trace 4 0/1 -> Motor current A history/1  "Motor iq A"
  Trace 3 0/1 -> Motor speed rpm history/1  "Motor speed rpm"
  Select 32/1 -> Nominal battery kWh/1
  Trace 7 0/1 -> Replenishment cost GHS history/1  "Electric refill GHS"
  Trace 7 1/1 -> Replenishment cost GHS history/2  "Diesel refill GHS"
  Select 3/1 -> SOC percent/1
  [results] -> Select 1/1
  [results] -> Select 10/1
  [results] -> Select 11/1
  [results] -> Select 12/1
  [results] -> Select 16/1
  [results] -> Select 17/1
  [results] -> Select 18/1
  [results] -> Select 2/1
  [results] -> Select 20/1
  [results] -> Select 21/1
  [results] -> Select 22/1
  [results] -> Select 23/1
  [results] -> Select 24/1
  [results] -> Select 25/1
  [results] -> Select 27/1
  [results] -> Select 28/1
  [results] -> Select 29/1
  [results] -> Select 3/1
  [results] -> Select 30/1
  [results] -> Select 31/1
  [results] -> Select 32/1
  [results] -> Select 33/1
  [results] -> Select 4/1
  [results] -> Select 5/1
  [results] -> Select 6/1
  [results] -> Select 7/1
  [results] -> Select 8/1
  [results] -> Select 9/1
  Select 1/1 -> Speed km per h/1
  [results] -> Trace 0 0/1
  [results] -> Trace 0 1/1
  [results] -> Trace 0 2/1
  [results] -> Trace 1 0/1
  [results] -> Trace 2 0/1
  [results] -> Trace 3 0/1
  [results] -> Trace 4 0/1
  [results] -> Trace 5 0/1
  [results] -> Trace 5 1/1
  [results] -> Trace 5 2/1
  [results] -> Trace 6 0/1
  [results] -> Trace 6 1/1
  [results] -> Trace 7 0/1
  [results] -> Trace 7 1/1
  [results] -> Trace 8 0/1
  Select 16/1 -> UNSERVED ELECTRIC DC kW/1
  results/1 -> [results]

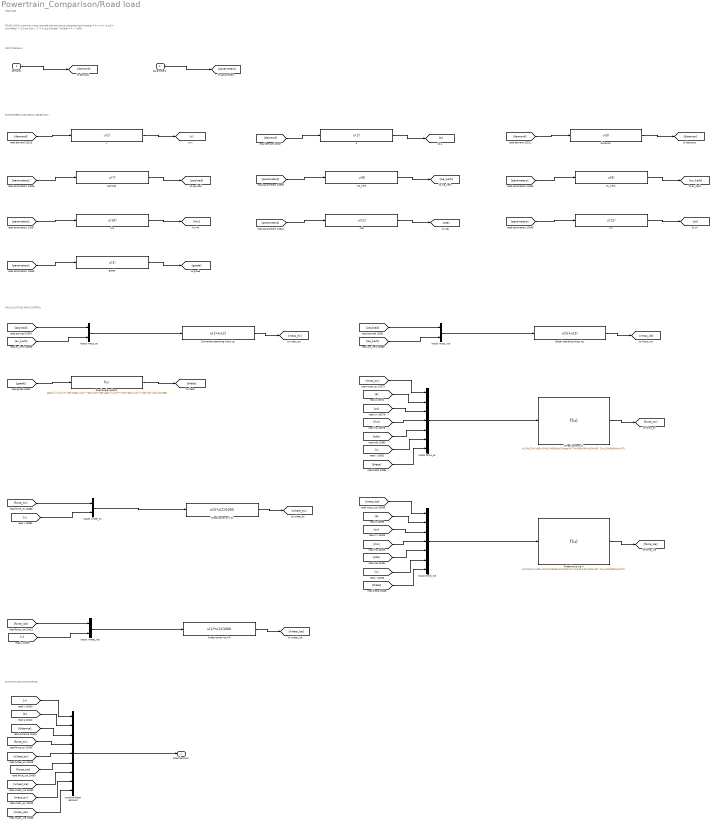
== system Powertrain_Comparison/Road load ==
  note: Road load
  note: ROAD LOAD | common route, payload and resistance; separate kerb masses
      | F = m a + m g Crr cos(theta) + 0.5 rho CdA v^2 + m g sin(theta). Pwheel = F v / 1000.
  note: INPUT SIGNALS
  note: PARAMETERS AND SIGNAL SELECTION
  note: CALCULATIONS AND CONTROL
  note: OUTPUTS AND MONITORING
  demand : Inport  PortDimensions=3
  parameters : Inport  Port=2  PortDimensions=52
  Converted operating mass kg : Fcn  Expr=u(1)+u(2)
  Diesel operating mass kg : Fcn  Expr=u(1)+u(2)
  Road angle radians : Fcn  Expr=atan((((((u(1))+(-20)+abs((u(1))-(-20)))/2)+(20)-abs((((u(1))+(-20)+abs((u(1))-(-20)))/2)-(20)))/2)/100)
  Wheel force ev N : Fcn  Expr=u(1)*u(2)+(u(6)>0)*u(1)*9.81*u(3)*cos(u(7))+0.5*u(4)*u(5)*u(6)^2+u(1)*9.81*sin(u(7))
  Wheel force ice N : Fcn  Expr=u(1)*u(2)+(u(6)>0)*u(1)*9.81*u(3)*cos(u(7))+0.5*u(4)*u(5)*u(6)^2+u(1)*9.81*sin(u(7))
  Wheel power ev kW : Fcn  Expr=u(1)*u(2)/1000
  Wheel power ice kW : Fcn  Expr=u(1)*u(2)/1000
  a : Fcn  Expr=u(2)
  cda : Fcn  Expr=u(11)
  combine Road demand : Mux  Inputs=9
  crr : Fcn  Expr=u(12)
  distance : Fcn  Expr=u(3)
  ev_kerb : Fcn  Expr=u(9)
  grade : Fcn  Expr=u(3)
  ice_kerb : Fcn  Expr=u(8)
  inputs force_ev : Mux  Inputs=7
  inputs force_ice : Mux  Inputs=7
  inputs mass_ev : Mux  Inputs=2
  inputs mass_ice : Mux  Inputs=2
  inputs wheel_ev : Mux  Inputs=2
  inputs wheel_ice : Mux  Inputs=2
  payload : Fcn  Expr=u(7)
  rho : Fcn  Expr=u(10)
  v : Fcn  Expr=u(1)
  Road demand : Outport  PortDimensions=9
  wires:
  [grade] -> Road angle radians/1
  [cda] -> inputs force_ice/5
  [v] -> inputs wheel_ev/2
  [force_ev] -> inputs wheel_ev/1
  distance/1 -> [distance]
  [wheel_ev] -> combine Road demand/5
  [demand] -> a/1
  Wheel power ev kW/1 -> [wheel_ev]
  [parameters] -> crr/1
  [parameters] -> cda/1
  [crr] -> inputs force_ice/3
  [v] -> inputs wheel_ice/2
  [force_ice] -> inputs wheel_ice/1
  [parameters] -> ev_kerb/1
  [parameters] -> rho/1
  parameters/1 -> [parameters]
  [mass_ev] -> inputs force_ev/1
  [rho] -> inputs force_ice/4
  [a] -> inputs force_ev/2
  [v] -> inputs force_ice/6
  [crr] -> inputs force_ev/3
  payload/1 -> [payload]
  v/1 -> [v]
  [rho] -> inputs force_ev/4
  [v] -> inputs force_ev/6
  [cda] -> inputs force_ev/5
  [a] -> inputs force_ice/2
  [theta] -> inputs force_ev/7
  [demand] -> v/1
  [v] -> combine Road demand/1
  [theta] -> inputs force_ice/7
  [a] -> combine Road demand/2
  [distance] -> combine Road demand/3
  [force_ev] -> combine Road demand/4
  [force_ice] -> combine Road demand/6
  [demand] -> distance/1
  [wheel_ice] -> combine Road demand/7
  [mass_ev] -> combine Road demand/8
  [mass_ice] -> combine Road demand/9
  [parameters] -> ice_kerb/1
  [payload] -> inputs mass_ev/1
  grade/1 -> [grade]
  [ev_kerb] -> inputs mass_ev/2
  a/1 -> [a]
  [payload] -> inputs mass_ice/1
  demand/1 -> [demand]
  [ice_kerb] -> inputs mass_ice/2
  [parameters] -> payload/1
  inputs force_ice/1 -> Wheel force ice N/1
  [mass_ice] -> inputs force_ice/1
  [parameters] -> grade/1
  Wheel power ice kW/1 -> [wheel_ice]
  inputs wheel_ev/1 -> Wheel power ev kW/1
  Road angle radians/1 -> [theta]
  crr/1 -> [crr]
  inputs wheel_ice/1 -> Wheel power ice kW/1
  cda/1 -> [cda]
  ev_kerb/1 -> [ev_kerb]
  rho/1 -> [rho]
  inputs force_ev/1 -> Wheel force ev N/1
  combine Road demand/1 -> Road demand/1
  ice_kerb/1 -> [ice_kerb]
  inputs mass_ev/1 -> Converted operating mass kg/1
  inputs mass_ice/1 -> Diesel operating mass kg/1
  Wheel force ev N/1 -> [force_ev]
  Converted operating mass kg/1 -> [mass_ev]
  Diesel operating mass kg/1 -> [mass_ice]
  Wheel force ice N/1 -> [force_ice]
